simulink model "ASM_Traffic"  (R2026a)
settings: Solver=ode1  StartTime=SIM.tstart.v  StopTime=SIM.tend.v  FixedStep=SIM.StepSize.v
PostLoadFcn:
  | if any(exist('dsrtsu_mdlpostloadfcn', 'file') ~= 0), dsrtsu_mdlpostloadfcn('Execute', bdroot); end
  | try, asm_mdl_postloadfcn(bdroot, 'UpdateModel', 3600); catch, disp(lasterr); end,
InitFcn:
  | , if any(exist('rtifpga_mdlclblib', 'file') ~= 0), rtifpga_mdlclblib('Init', bdroot); end,
  | , if any(exist('dsmpb_private', 'file') ~= 0), dsmpb_private('dsmpb_mdlclblib', 'Init', bdroot); end,
model workspace (MAT data in the model file):
  asmReferencePath = [0 0.01 0.02 0.03 0.04 0.05 0.06 0.07 0.08 0.09 0.1 0.11 ... (350007 elements, 50001x7)]
  roadBounds : Simulink.Parameter (value not decoded)
  safetyAxes : Simulink.Parameter (value not decoded)
undefined symbols (not defined in the file): _to_, a0b2, ASM_BrakeHydraulics_DemoSystems, ASM_VehicleDynamics_DemoSystems, b98103fe8ad365046cd0, BrakeCircuit, controllerConfig, CPT, Crankshaft, DiscIntNeverNeededParam, dsmsi, FinalDriveAssembly, MDL, ModeSignals, mu, Pos_BrakePedal_Maneuver, rad, RefSignals, roadFamilyData, roadFamilyId, s_to_rpm, SIM, SoftECU, Suspension, Tire, Transmission
libraries: ASM_Traffic_lib x135, simulink x98, ASM_Utils_lib x77, ASM_VehicleDynamics_lib x70, ASM_Environment_lib x22, dsmpblib x20, dsmsilib x15, MDLD_Utils_lib x10, ASM_BrakeHydraulics_lib x3, sl_discontinuities x2
(part 11 of 65)

== system ASM_Traffic/DomainControl/DriverAssistance/Interface_In ==
  note: Driver Assistance
  In : Inport
  Bus Creator : BusCreator  Inputs=2
  Bus Selector : BusSelector  OutputSignals=Environment.Plant.Sw_ModelPortBlocks[0Disabled|1Enabled],Environment.Plant.Sw_ModelDeskPlottingInterface[0Disabled|1Enabled],VehicleDynamics.Plant.v_x_Vehicle_CoG[km|h],VehicleDynamics.Plant.YawRate_Vehicle_CoG[deg|s],VehicleDynamics.Plant.Pos_FL_Wheel[x;y;z][m],VehicleDynamics.Plant.Pos_FR_Wheel[x;y;z][m],VehicleDynamics.Plant.r_Dyn_Tire[FL;FR;RL;RR][m],VehicleDynamics.Plant.Coef_RollingRes[FL;FR;RL;RR][],VehicleDynamics.Plant.Cw_x[],VehicleDynamics.Plant.m_TotalVehicle[kg],Drivetrain.Plant.i_FrontDrive[],Drivetrain.Plant.i_RearDrive[],Drivetrain.Plant.TrqDistri_Front_Rear[0_1],Drivetrain.Plant.i_unsync_Trm[],Driver.Plant.Pos_AccPedal[%],Driver.Plant.Pos_BrakePedal[%],Environment.Plant.Slope_Veh_Road[%],Environment.Plant.s_Vehicle_Road[m],Environment.Plant.d_Vehicle_Road[m],Environment.Plant.ECU_Commands[],Environment.Plant.Reset_States[0|1],Environment.Plant.Dist_Fellows[m],Environment.Plant.v_Rel_Fellows[m|s],Environment.Plant.Angle_Hor_Rel_Fellows[deg],Environment.Plant.s_Fellows_Ref[m],Environment.Plant.d_Total_Fellows[m],Environment.Plant.PosVec_MainPnt_Fellows[x;y;z][m],Environment.Plant.Length_Fellows[m],Environment.Plant.Width_Fellows[m],Environment.Plant.Height_Fellows[m],Environment.Plant.Object_ID[],VehicleDynamics.Plant.v_Vehicle[km|h],Engine.Plant.Trq_Fric_Engine[Nm]
  Bus Selector1 : BusSelector  OutputSignals=Environment.Plant.Sw_ModelPortBlocks[0Disabled|1Enabled]
  ExternalSignals : Subsystem
  ModelSignals : Subsystem
  Out : Outport  VectorParamsAs1DForOutWhenUnconnected=off
  wires:
  Bus Selector1/1 -> ExternalSignals/Enable  "<Sw_ModelPortBlocks[0Disabled|1Enabled]>"
  ExternalSignals/1(ExternalECU_ACC_Out) -> Bus Creator/2
  Bus Selector/2 -> ModelSignals/2(Sw_ModelDeskPlottingInterface[0Disabled|1Enabled])  "<Sw_ModelDeskPlottingInterface[0Disabled|1Enabled]>"
  Bus Selector/1 -> ModelSignals/1(Sw_ModelPortBlocks[0Disabled|1Enabled])  "<Sw_ModelPortBlocks[0Disabled|1Enabled]>"
  In/1 -> Bus Selector1/1, Bus Selector/1
  Bus Selector/32 -> ModelSignals/32(v_Vehicle[km|h])  "<v_Vehicle[km|h]>"
  ModelSignals/1(Out) -> Bus Creator/1
  Bus Selector/31 -> ModelSignals/31(Object_ID[])  "<Object_ID[]>"
  Bus Selector/30 -> ModelSignals/30(Height_Fellows[m])  "<Height_Fellows[m]>"
  Bus Selector/29 -> ModelSignals/29(Width_Fellows[m])  "<Width_Fellows[m]>"
  Bus Selector/28 -> ModelSignals/28(Length_Fellows[m])  "<Length_Fellows[m]>"
  Bus Selector/27 -> ModelSignals/27(PosVec_MainPnt_Fellows[x;y;z][m])  "<PosVec_MainPnt_Fellows[x;y;z][m]>"
  Bus Selector/26 -> ModelSignals/26(d_Total_Fellows[m])  "<d_Total_Fellows[m]>"
  Bus Selector/25 -> ModelSignals/25(s_Fellows_Ref[m])  "<s_Fellows_Ref[m]>"
  Bus Selector/24 -> ModelSignals/24(Angle_Hor_Rel_Fellows[deg])  "<Angle_Hor_Rel_Fellows[deg]>"
  Bus Selector/23 -> ModelSignals/23(v_Rel_Fellows[m|s])  "<v_Rel_Fellows[m|s]>"
  Bus Selector/22 -> ModelSignals/22(Dist_Fellows[m])  "<Dist_Fellows[m]>"
  Bus Selector/21 -> ModelSignals/21(Reset[0|1])  "<Reset_States[0|1]>"
  Bus Selector/20 -> ModelSignals/20(ECU_Commands[])  "<ECU_Commands[]>"
  Bus Selector/19 -> ModelSignals/19(d_Vehicle_Road[m])  "<d_Vehicle_Road[m]>"
  Bus Selector/18 -> ModelSignals/18(s_Vehicle_Road[m])  "<s_Vehicle_Road[m]>"
  Bus Selector/17 -> ModelSignals/17(Slope_Veh_Road[%])  "<Slope_Veh_Road[%]>"
  Bus Selector/16 -> ModelSignals/16(Pos_BrakePedal[%])  "<Pos_BrakePedal[%]>"
  Bus Selector/15 -> ModelSignals/15(Pos_AccPedal[%])  "<Pos_AccPedal[%]>"
  Bus Selector/11 -> ModelSignals/11(i_FrontDrive[])  "<i_FrontDrive[]>"
  Bus Selector/10 -> ModelSignals/10(m_TotalVehicle[kg])  "<m_TotalVehicle[kg]>"
  Bus Selector/9 -> ModelSignals/9(Cw_x[])  "<Cw_x[]>"
  Bus Selector/8 -> ModelSignals/8(Coef_RollingRes[FL;FR;RL;RR][])  "<Coef_RollingRes[FL;FR;RL;RR][]>"
  Bus Selector/7 -> ModelSignals/7(r_Dyn_Tire[FL;FR;RL;RR][m])  "<r_Dyn_Tire[FL;FR;RL;RR][m]>"
  Bus Selector/6 -> ModelSignals/6(Pos_FR_Wheel[x;y;z][m])  "<Pos_FR_Wheel[x;y;z][m]>"
  Bus Selector/5 -> ModelSignals/5(Pos_FL_Wheel[x;y;z][m])  "<Pos_FL_Wheel[x;y;z][m]>"
  Bus Selector/4 -> ModelSignals/4(YawRate_Vehicle_CoG[deg|s])  "<YawRate_Vehicle_CoG[deg|s]>"
  Bus Selector/3 -> ModelSignals/3(v_x_Vehicle_CoG[km|h])  "<v_x_Vehicle_CoG[km|h]>"
  Bus Creator/1 -> Out/1
  Bus Selector/14 -> ModelSignals/14(i_unsync_Trm[])  "<i_unsync_Trm[]>"
  Bus Selector/33 -> ModelSignals/33(Trq_Fric_Engine[Nm])  "<Trq_Fric_Engine[Nm]>"
  Bus Selector/12 -> ModelSignals/12(i_RearDrive[])  "<i_RearDrive[]>"
  Bus Selector/13 -> ModelSignals/13(TrqDistri_Front_Rear[0_1][])  "<TrqDistri_Front_Rear[0_1]>"

== system ASM_Traffic/DomainControl/DriverAssistance/Interface_Out ==
  note: Driver Assistance
  In : Inport
  Animation : Subsystem
  Bus Creator1 : BusCreator  Inputs=2
  Bus Selector5 : BusSelector  OutputSignals=SoftECU_ACC.Controller_ACC.State_ACC[0Off|1On],SoftECU_ACC.Target_Selection_ACC.Target_Detected[0|1],SoftECU_ACC.Controller_ACC.v_Set[km|h],SoftECU_ACC.Controller_ACC.Distance_Set[m],SoftECU_ACC.Target_Selection_ACC.Dist_Long[m]
  Bus Selector6 : BusSelector  OutputSignals=ECU_ACC.Enable_Trq_Increase_ACC[0|1],ECU_ACC.Trq_IncreaseRequest_ACC[Nm],ECU_ACC.Trq_IncreaseRequest_ACC[Front;Rear][Nm],ECU_ACC.Enable_Trq_Decrease_ACC[0|1],ECU_ACC.Trq_DecreaseRequest_ACC[Nm],ECU_ACC.AEB[0|1],ECU_ACC.FCW[0|1],ECU_ACC.ACC_State[1OFF|2Standby|3ON],ECU_ACC.Driver_Override_ACC_Active[0Off|1On],ECU_ACC.Driver_Override_ACC_Reason[0NoOverride|1BrakePedal|2AccPedal]
  Control_ModelSignals : Subsystem
  Out : Outport  VectorParamsAs1DForOutWhenUnconnected=off
  wires:
  Bus Selector6/6 -> Control_ModelSignals/6(AEB[0|1])  "<AEB[0|1]>"
  Bus Selector6/7 -> Control_ModelSignals/7(FCW[0|1])  "<FCW[0|1]>"
  Bus Selector6/5 -> Control_ModelSignals/5(Trq_DecreaseRequest_ACC[Nm])  "<Trq_DecreaseRequest_ACC[Nm]>"
  Bus Selector6/4 -> Control_ModelSignals/4(Enable_Trq_Decrease_ACC[0|1])  "<Enable_Trq_Decrease_ACC[0|1]>"
  Bus Selector6/2 -> Control_ModelSignals/2(Trq_IncreaseRequest_ACC[Nm])  "<Trq_IncreaseRequest_ACC[Nm]>"
  Bus Selector6/1 -> Control_ModelSignals/1(Enable_Trq_Increase_ACC[0|1])  "<Enable_Trq_Increase_ACC[0|1]>"
  In/1 -> Bus Selector5/1, Bus Selector6/1
  Bus Selector6/3 -> Control_ModelSignals/3(Trq_IncreaseRequest_ACC[Front;Rear][Nm])  "<Trq_IncreaseRequest_ACC[Front;Rear][Nm]>"
  Bus Creator1/1 -> Out/1  "DriverAssistance"
  Control_ModelSignals/1(Out) -> Bus Creator1/1
  Animation/1(Out) -> Bus Creator1/2
  Bus Selector5/1 -> Animation/1(State_ACC[0Off|1On])  "<State_ACC[0Off|1On]>"
  Bus Selector5/2 -> Animation/2(Target_Detected[0|1])  "<Target_Detected[0|1]>"
  Bus Selector5/3 -> Animation/3(v_Set[km|h])  "<v_Set[km|h]>"
  Bus Selector5/4 -> Animation/4(Distance_Set[m])  "<Distance_Set[m]>"
  Bus Selector5/5 -> Animation/5(Dist_Long[m])  "<Dist_Long[m]>"
  Bus Selector6/8 -> Control_ModelSignals/8(ACC_State[1OFF|2Standby|3ON])  "<ACC_State[1OFF|2Standby|3ON]>"
  Bus Selector6/9 -> Control_ModelSignals/9(Driver_Override_ACC_Active[0Off|1On])  "<Driver_Override_ACC_Active[0Off|1On]>"
  Bus Selector6/10 -> Control_ModelSignals/10(Driver_Override_ACC_Reason[0NoOverride|1BrakePedal|2AccPedal])  "<Driver_Override_ACC_Reason[0NoOverride|1BrakePedal|2AccPedal]>"

== system ASM_Traffic/DomainControl/DriverAssistance/SignalInterface ==
  In : Inport
  ASMSignalInterface : Subsystem  mask(ASM_SIGNAL_INTERFACE){LabelTextfield=DriverAssistance}
      mask prompts: LabelTextfield "Label"
      mask help:
      | The ASMSignalInterface block processes the ASMSignalBus and provides a vector-based interface for each signal (e.g. ModelDesk Plotting).
      |
      | Always push the update button after you have changed the signal bus structure in order to synchronize the signal interface. The update may take a few seconds.
      | A modified model must be reloaded in ModelDesk to keep consistency of ModelDesk and simulation model plot signals. Therefore select ''Update Model'' from the ''Simulation Model'' context menu of the ModelDesk Project Navigator.
      settings: AttributesFormatString=Label: %<LabelTextfield>
      settings: CopyFcn=|
      | try
      |  set_param(gcb,'LinkStatus', 'none')
      | catch
      | end
      mask Help: eval(['asm_modelhelp(gcbh,''tool'',''ASM_Utils_lib'', ''ASMSIGNALINTERFACE'')'])
      mask DialogControl Hint Prompt: For changes of Label first apply change and then push "Update".
      mask DialogControl UpdateButton Prompt: Update
      mask DialogControl UpdateButton Callback: asm_mdld_plot_block_update(bdroot(gcb), 'update', 'current');
      mask DialogControl UpdateAllButton Prompt: Update All
      mask DialogControl UpdateAllButton Callback: asm_mdld_plot_block_update(bdroot(gcb), 'update', 'all');
  Bus Selector Disable Signals : BusSelector  OutputSignals=ExternalModel.Sw_ModelPortBlocks[0Disabled|1Enabled],ExternalModel.Sw_ModelDeskPlottingInterface[0Disabled|1Enabled]
  ExternalOutports : Subsystem  TreatAsAtomicUnit=on
  wires:
  Bus Selector Disable Signals/2 -> ASMSignalInterface/Enable  "<Sw_ModelDeskPlottingInterface[0Disabled|1Enabled]>"
  Bus Selector Disable Signals/1 -> ExternalOutports/Enable  "<Sw_ModelPortBlocks[0Disabled|1Enabled]>"
  In/1 -> Bus Selector Disable Signals/1
  [ASMBUS_DriverAssistance_Control] -> ASMSignalInterface/1(ASMSignalBus), ExternalOutports/1(In1)

== system ASM_Traffic/DomainControl/StartSystem/Control ==
  note: Start System
  Interface_In : Inport
  SoftECU_StartSystem : Subsystem
  Sw_ECU_Signals : Subsystem
  UserInterface : Subsystem
  Control : Outport  VectorParamsAs1DForOutWhenUnconnected=off
  wires:
  SoftECU_StartSystem/1(ASMSignalBus) -> UserInterface/2(In)
  UserInterface/1(Out) -> SoftECU_StartSystem/1(UserInterface)
  Interface_In/1 -> Sw_ECU_Signals/2(ExternalECU), SoftECU_StartSystem/2(Interface_In), UserInterface/1(Interface_In)
  Sw_ECU_Signals/1(ECU_Signals) -> Control/1
  SoftECU_StartSystem/2(Out) -> Sw_ECU_Signals/1(SoftECU)

== system ASM_Traffic/DomainControl/StartSystem/Interface_In ==
  note: Start System
  In : Inport
  Bus Creator : BusCreator  Inputs=2
  Bus Selector2 : BusSelector  OutputSignals=Environment.Plant.Sw_ModelPortBlocks[0Disabled|1Enabled],Environment.Plant.Sw_ModelDeskPlottingInterface[0Disabled|1Enabled],Driver.Plant.Pos_BrakePedal[%],Driver.Plant.Pos_ClutchPedal[%],Driver.Plant.SelectorLever[-3T|-2P|-1R|0N|1D],Environment.Plant.Reset_States[0|1],Environment.Plant.Sw_StartButton[0Off|1On],DomainControl.TorqueManager.Control.State_Engine[0|1|2|3|4],Environment.Plant.State_StartButton[-1PowerOff|0Acc|1PowerOn|2StarterOn],Drivetrain.Plant.Mode_Transmission[1Manual|2Automatic],Drivetrain.Plant.Sw_CrankShaft_Reset[0Disabled|1Enabled],Environment.Plant.Mode_StartButtonState[1Stim|2SoftECU]
  Bus Selector21 : BusSelector  OutputSignals=Environment.Plant.Sw_ModelPortBlocks[0Disabled|1Enabled]
  ExternalSignals : Subsystem
  ModelSignals : Subsystem
  Out : Outport  VectorParamsAs1DForOutWhenUnconnected=off
  wires:
  Bus Selector21/1 -> ExternalSignals/Enable  "<Sw_ModelPortBlocks[0Disabled|1Enabled]>"
  ExternalSignals/1(ExternalECU_StartSystem_Out) -> Bus Creator/2
  Bus Selector2/2 -> ModelSignals/2(Sw_ModelDeskPlottingInterface[0Disabled|1Enabled])  "<Sw_ModelDeskPlottingInterface[0Disabled|1Enabled]>"
  Bus Selector2/1 -> ModelSignals/1(Sw_ModelPortBlocks[0Disabled|1Enabled])  "<Sw_ModelPortBlocks[0Disabled|1Enabled]>"
  In/1 -> Bus Selector21/1, Bus Selector2/1
  Bus Selector2/7 -> ModelSignals/7(Sw_StartButton[0Off|1On])  "<Sw_StartButton[0Off|1On]>"
  Bus Creator/1 -> Out/1
  Bus Selector2/6 -> ModelSignals/6(Reset_States[0|1])  "<Reset_States[0|1]>"
  Bus Selector2/5 -> ModelSignals/5(SelectorLever[-3T|-2P|-1R|0N|1D])  "<SelectorLever[-3T|-2P|-1R|0N|1D]>"
  Bus Selector2/3 -> ModelSignals/3(Pos_BrakePedal[%])  "<Pos_BrakePedal[%]>"
  Bus Selector2/4 -> ModelSignals/4(Pos_ClutchPedal[%])  "<Pos_ClutchPedal[%]>"
  Bus Selector2/8 -> ModelSignals/8(State_Engine[0|1|2|3|4])  "<State_Engine[0|1|2|3|4]>"
  Bus Selector2/9 -> ModelSignals/9(State_StartButton[-1PowerOff|0Acc|1PowerOn|2StarterOn])  "<State_StartButton[-1PowerOff|0Acc|1PowerOn|2StarterOn]>"
  Bus Selector2/10 -> ModelSignals/10(Mode_Transmission[1Manual|2Automatic])  "<Mode_Transmission[1Manual|2Automatic]>"
  Bus Selector2/11 -> ModelSignals/11(Sw_CrankShaft_Reset[0Disabled|1Enabled])  "<Sw_CrankShaft_Reset[0Disabled|1Enabled]>"
  Bus Selector2/12 -> ModelSignals/12(Mode_StartButtonState[1Stim|2SoftECU])  "<Mode_StartButtonState[1Stim|2SoftECU]>"
  ModelSignals/1(Out) -> Bus Creator/1

== system ASM_Traffic/DomainControl/StartSystem/Interface_Out ==
  note: Start System
  In : Inport
  Bus Creator1 : BusCreator  Inputs=1
  Bus Selector1 : BusSelector  OutputSignals=State_StartButton[-2|-1|0|1|2|3],Sw_Ignition[0|1],Sw_StarterReq[0|1]
  Control_ModelSignals : Subsystem
  Out : Outport  VectorParamsAs1DForOutWhenUnconnected=off
  wires:
  In/1 -> Bus Selector1/1
  Bus Selector1/2 -> Control_ModelSignals/2(Sw_Ignition[0|1])  "<Sw_Ignition[0|1]>"
  Bus Selector1/3 -> Control_ModelSignals/3(Sw_StarterReq[0|1])  "<Sw_StarterReq[0|1]>"
  Bus Creator1/1 -> Out/1  "StartSystem"
  Control_ModelSignals/1(Out) -> Bus Creator1/1
  Bus Selector1/1 -> Control_ModelSignals/1(State_StartButton[-2|-1|0|1|2|3])  "<State_StartButton[-2|-1|0|1|2|3]>"

== system ASM_Traffic/DomainControl/StartSystem/SignalInterface ==
  In : Inport
  ASMSignalInterface : Subsystem  mask(ASM_SIGNAL_INTERFACE){LabelTextfield=StartSystem}
      mask prompts: LabelTextfield "Label"
      mask help:
      | The ASMSignalInterface block processes the ASMSignalBus and provides a vector-based interface for each signal (e.g. ModelDesk Plotting).
      |
      | Always push the update button after you have changed the signal bus structure in order to synchronize the signal interface. The update may take a few seconds.
      | A modified model must be reloaded in ModelDesk to keep consistency of ModelDesk and simulation model plot signals. Therefore select ''Update Model'' from the ''Simulation Model'' context menu of the ModelDesk Project Navigator.
      settings: AttributesFormatString=Label: %<LabelTextfield>
      settings: CopyFcn=|
      | try
      |  set_param(gcb,'LinkStatus', 'none')
      | catch
      | end
      mask Help: eval(['asm_modelhelp(gcbh,''tool'',''ASM_Utils_lib'', ''ASMSIGNALINTERFACE'')'])
      mask DialogControl Hint Prompt: For changes of Label first apply change and then push "Update".
      mask DialogControl UpdateButton Prompt: Update
      mask DialogControl UpdateButton Callback: asm_mdld_plot_block_update(bdroot(gcb), 'update', 'current');
      mask DialogControl UpdateAllButton Prompt: Update All
      mask DialogControl UpdateAllButton Callback: asm_mdld_plot_block_update(bdroot(gcb), 'update', 'all');
  Bus Selector Disable Signals : BusSelector  OutputSignals=ExternalModel.Sw_ModelPortBlocks[0Disabled|1Enabled],ExternalModel.Sw_ModelDeskPlottingInterface[0Disabled|1Enabled]
  ExternalOutports : Subsystem  TreatAsAtomicUnit=on
  wires:
  Bus Selector Disable Signals/2 -> ASMSignalInterface/Enable  "<Sw_ModelDeskPlottingInterface[0Disabled|1Enabled]>"
  Bus Selector Disable Signals/1 -> ExternalOutports/Enable  "<Sw_ModelPortBlocks[0Disabled|1Enabled]>"
  In/1 -> Bus Selector Disable Signals/1
  [ASMBUS_StartSystem_Control] -> ASMSignalInterface/1(ASMSignalBus), ExternalOutports/1(In1)

== system ASM_Traffic/DomainControl/TorqueManager/Control ==
  note: Torque Manager Basic
  Interface_In : Inport
  SoftECU_TorqueManager : Subsystem
  UserInterface : Subsystem
  Control : Outport  VectorParamsAs1DForOutWhenUnconnected=off
  wires:
  SoftECU_TorqueManager/1(ASMSignalBus) -> UserInterface/1(In)
  UserInterface/1(Out) -> SoftECU_TorqueManager/1(UserInterface)
  Interface_In/1 -> SoftECU_TorqueManager/2(Interface_In)
  SoftECU_TorqueManager/2(Out) -> Control/1

== system ASM_Traffic/DomainControl/TorqueManager/Interface_In ==
  note: Torque Manager Basic
  In : Inport
  Bus Creator : BusCreator  Inputs=1
  Bus Selector2 : BusSelector  OutputSignals=Environment.Plant.Sw_ModelPortBlocks[0Disabled|1Enabled],Environment.Plant.Sw_ModelDeskPlottingInterface[0Disabled|1Enabled],Driver.Plant.Pos_BrakePedal[%],Engine.Control.State_ICEngine[0|1|2|3|4],DomainControl.StartSystem.Control.Sw_Ignition[0|1],DomainControl.StartSystem.Control.Sw_StarterReq[0|1],Engine.Control.Sw_Starter[0Off|1On]
  ModelSignals : Subsystem
  Out : Outport  VectorParamsAs1DForOutWhenUnconnected=off
  wires:
  Bus Selector2/2 -> ModelSignals/2(Sw_ModelDeskPlottingInterface[0Disabled|1Enabled])  "<Sw_ModelDeskPlottingInterface[0Disabled|1Enabled]>"
  Bus Selector2/1 -> ModelSignals/1(Sw_ModelPortBlocks[0Disabled|1Enabled])  "<Sw_ModelPortBlocks[0Disabled|1Enabled]>"
  In/1 -> Bus Selector2/1
  Bus Selector2/4 -> ModelSignals/4(State_Engine[0|1|2|3|4])  "<State_ICEngine[0|1|2|3|4]>"
  Bus Selector2/3 -> ModelSignals/3(Pos_BrakePedal[%])  "<Pos_BrakePedal[%]>"
  ModelSignals/1(Out) -> Bus Creator/1
  Bus Creator/1 -> Out/1
  Bus Selector2/5 -> ModelSignals/5(Sw_Ignition[0|1])  "<Sw_Ignition[0|1]>"
  Bus Selector2/6 -> ModelSignals/6(Sw_StarterReq[0|1])  "<Sw_StarterReq[0|1]>"
  Bus Selector2/7 -> ModelSignals/7(Sw_Starter[0Off|1On])  "<Sw_Starter[0Off|1On]>"

== system ASM_Traffic/DomainControl/TorqueManager/Interface_Out ==
  note: Torque Manager Basic
  In : Inport
  " Mode_BSG[-1|0|1|2|3|4|5]" : Constant  Value=-1
  Bus Creator1 : BusCreator  Inputs=1
  Bus Selector : BusSelector  OutputSignals=ExternalModel.Sw_Ignition[0|1],ExternalModel.Sw_StarterReq[0|1],ExternalModel.Pos_BrakePedal[%],ExternalModel.Sw_Starter[0Off|1On],ExternalModel.State_Engine[0|1|2|3|4]
  Control_ModelSignals : Subsystem
  HybridMode_ICE[0Off|1OnIdle|2OnPower|3err] : Constant  Value=0
  Sw_DriveMode[0Hybrid|1ICE|2EM] : Constant
  Trq_Request_Brake[Nm] : Constant  Value=0
  Trq_Request_EM[Nm] : Constant  Value=0
  Trq_Request_ICE[Nm] : Constant  Value=-9000
  Vehicle_Topology[-2|-1|0|2] : Constant  Value=-1
  Out : Outport  VectorParamsAs1DForOutWhenUnconnected=off
  wires:
  HybridMode_ICE[0Off|1OnIdle|2OnPower|3err]/1 -> Control_ModelSignals/9(HybridMode_ICE[0Off|1OnIdle|2OnPower|3err])
  Trq_Request_ICE[Nm]/1 -> Control_ModelSignals/8(Trq_Request_ICE[Nm])
  Sw_DriveMode[0Hybrid|1ICE|2EM]/1 -> Control_ModelSignals/11(Sw_DriveMode[0Hybrid|1ICE|2EM])
  In/1 -> Bus Selector/1
  Control_ModelSignals/1(Out) -> Bus Creator1/1
  Bus Selector/1 -> Control_ModelSignals/1(Ignition_ICE[0Off|1On])  "<Sw_Ignition[0|1]>"
  Bus Selector/2 -> Control_ModelSignals/2(StarterReq_ICE[0Off|1On])  "<Sw_StarterReq[0|1]>"
  Bus Selector/3 -> Control_ModelSignals/3(Pos_BrakePedal_Desired[%])  "<Pos_BrakePedal[%]>"
  Trq_Request_EM[Nm]/1 -> Control_ModelSignals/7(Trq_Request_EM[Nm])
  " Mode_BSG[-1|0|1|2|3|4|5]"/1 -> Control_ModelSignals/6(" Mode_BSG[-1|0|1|2|3|4|5]")
  Bus Selector/4 -> Control_ModelSignals/4(Starter_Drivetrain[0Off|1On])  "<Sw_Starter[0Off|1On]>"
  Trq_Request_Brake[Nm]/1 -> Control_ModelSignals/10(Trq_Request_Brake[Nm])
  Vehicle_Topology[-2|-1|0|2]/1 -> Control_ModelSignals/12(Vehicle_Topology[-2|-1|0|2])
  Bus Creator1/1 -> Out/1  "TorqueManager"
  Bus Selector/5 -> Control_ModelSignals/5(State_Engine[0|1|2|3|4])  "<State_Engine[0|1|2|3|4]>"

== system ASM_Traffic/DomainControl/TorqueManager/SignalInterface ==
  In : Inport
  ASMSignalInterface : Subsystem  mask(ASM_SIGNAL_INTERFACE){LabelTextfield=TorqueManager}
      mask prompts: LabelTextfield "Label"
      mask help:
      | The ASMSignalInterface block processes the ASMSignalBus and provides a vector-based interface for each signal (e.g. ModelDesk Plotting).
      |
      | Always push the update button after you have changed the signal bus structure in order to synchronize the signal interface. The update may take a few seconds.
      | A modified model must be reloaded in ModelDesk to keep consistency of ModelDesk and simulation model plot signals. Therefore select ''Update Model'' from the ''Simulation Model'' context menu of the ModelDesk Project Navigator.
      settings: AttributesFormatString=Label: %<LabelTextfield>
      settings: CopyFcn=|
      | try
      |  set_param(gcb,'LinkStatus', 'none')
      | catch
      | end
      mask Help: eval(['asm_modelhelp(gcbh,''tool'',''ASM_Utils_lib'', ''ASMSIGNALINTERFACE'')'])
      mask DialogControl Hint Prompt: For changes of Label first apply change and then push "Update".
      mask DialogControl UpdateButton Prompt: Update
      mask DialogControl UpdateButton Callback: asm_mdld_plot_block_update(bdroot(gcb), 'update', 'current');
      mask DialogControl UpdateAllButton Prompt: Update All
      mask DialogControl UpdateAllButton Callback: asm_mdld_plot_block_update(bdroot(gcb), 'update', 'all');
  Bus Selector Disable Signals : BusSelector  OutputSignals=ExternalModel.Sw_ModelPortBlocks[0Disabled|1Enabled],ExternalModel.Sw_ModelDeskPlottingInterface[0Disabled|1Enabled]
  ExternalOutports : Subsystem  TreatAsAtomicUnit=on
  wires:
  Bus Selector Disable Signals/2 -> ASMSignalInterface/Enable  "<Sw_ModelDeskPlottingInterface[0Disabled|1Enabled]>"
  Bus Selector Disable Signals/1 -> ExternalOutports/Enable  "<Sw_ModelPortBlocks[0Disabled|1Enabled]>"
  In/1 -> Bus Selector Disable Signals/1
  [ASMBUS_TorqueManager_Control] -> ExternalOutports/1(In1), ASMSignalInterface/1(ASMSignalBus)

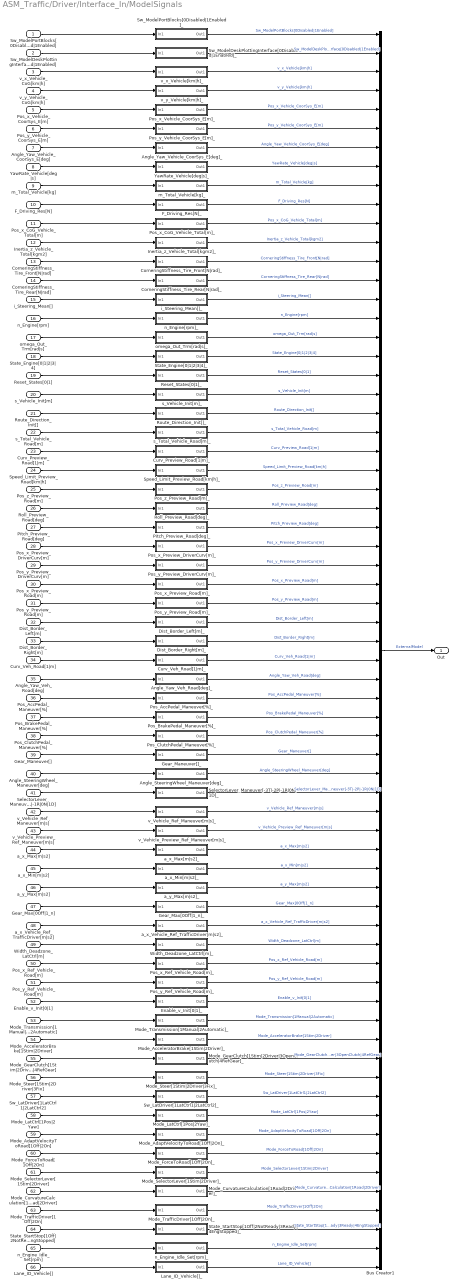
== system ASM_Traffic/Driver/Interface_In/ModelSignals ==
  Sw_ModelPortBlocks[0Disabled|1Enabled] : Inport
  Sw_ModelDeskPlottingInterface[0Disabled|1Enabled] : Inport  Port=2
  v_x_Vehicle_CoG[km|h] : Inport  Port=3
  v_y_Vehicle_CoG[km|h] : Inport  Port=4
  Pos_x_Vehicle_CoorSys_E[m] : Inport  Port=5
  Pos_y_Vehicle_CoorSys_E[m] : Inport  Port=6
  Angle_Yaw_Vehicle_CoorSys_E[deg] : Inport  Port=7
  YawRate_Vehicle[deg|s] : Inport  Port=8
  m_Total_Vehicle[kg] : Inport  Port=9
  F_Driving_Res[N] : Inport  Port=10
  Pos_x_CoG_Vehicle_Total[m] : Inport  Port=11
  Inertia_z_Vehicle_Total[kgm2] : Inport  Port=12
  CorneringStiffness_Tire_Front[N|rad] : Inport  Port=13
  CorneringStiffness_Tire_Rear[N|rad] : Inport  Port=14
  i_Steering_Mean[] : Inport  Port=15
  n_Engine[rpm] : Inport  Port=16
  omega_Out_Trm[rad|s] : Inport  Port=17
  State_Engine[0|1|2|3|4] : Inport  Port=18
  Reset_States[0|1] : Inport  Port=19
  s_Vehicle_Init[m] : Inport  Port=20
  Route_Direction_Init[] : Inport  Port=21
  s_Total_Vehicle_Road[m] : Inport  Port=22
  Curv_Preview_Road[1|m] : Inport  Port=23
  Speed_Limit_Preview_Road[km|h] : Inport  Port=24
  Pos_z_Preview_Road[m] : Inport  Port=25
  Roll_Preview_Road[deg] : Inport  Port=26
  Pitch_Preview_Road[deg] : Inport  Port=27
  Pos_x_Preview_DriverCurv[m] : Inport  Port=28
  Pos_y_Preview_DriverCurv[m] : Inport  Port=29
  Pos_x_Preview_Road[m] : Inport  Port=30
  Pos_y_Preview_Road[m] : Inport  Port=31
  Dist_Border_Left[m] : Inport  Port=32
  Dist_Border_Right[m] : Inport  Port=33
  Curv_Veh_Road[1|m] : Inport  Port=34
  Angle_Yaw_Veh_Road[deg] : Inport  Port=35
  Pos_AccPedal_Maneuver[%] : Inport  Port=36
  Pos_BrakePedal_Maneuver[%] : Inport  Port=37
  Pos_ClutchPedal_Maneuver[%] : Inport  Port=38
  Gear_Maneuver[] : Inport  Port=39
  Angle_SteeringWheel_Maneuver[deg] : Inport  Port=40
  SelectorLever_Maneuver[-3T|-2P|-1R|0N|1D] : Inport  Port=41
  v_Vehicle_Ref_Maneuver[m|s] : Inport  Port=42
  v_Vehicle_Preview_Ref_Maneuver[m|s] : Inport  Port=43
  a_x_Max[m|s2] : Inport  Port=44
  a_x_Min[m|s2] : Inport  Port=45
  a_y_Max[m|s2] : Inport  Port=46
  Gear_Max[0Off|1_n] : Inport  Port=47
  a_x_Vehicle_Ref_TrafficDriver[m|s2] : Inport  Port=48
  Width_Deadzone_LatCtrl[m] : Inport  Port=49
  Pos_x_Ref_Vehicle_Road[m] : Inport  Port=50
  Pos_y_Ref_Vehicle_Road[m] : Inport  Port=51
  Enable_v_Init[0|1] : Inport  Port=52
  Mode_Transmission[1Manual|2Automatic] : Inport  Port=53
  Mode_AcceleratorBrake[1Stim|2Driver] : Inport  Port=54
  Mode_GearClutch[1Stim|2Driver|3OpenClutch|4RefGear] : Inport  Port=55
  Mode_Steer[1Stim|2Driver|3Fix] : Inport  Port=56
  Sw_LatDriver[1LatCtrl1|2LatCtrl2] : Inport  Port=57
  Mode_LatCtrl[1Pos|2Yaw] : Inport  Port=58
  Mode_AdaptVelocityToRoad[1Off|2On] : Inport  Port=59
  Mode_ForceToRoad[1Off|2On] : Inport  Port=60
  Mode_SelectorLever[1Stim|2Driver] : Inport  Port=61
  Mode_CurvatureCalculation[1Road|2Driver] : Inport  Port=62
  Mode_TrafficDriver[1Off|2On] : Inport  Port=63
  State_StartStop[1Off|2NotReady|3Ready|4EngStopped] : Inport  Port=64
  n_Engine_Idle_Set[rpm] : Inport  Port=65
  Lane_ID_Vehicle[] : Inport  Port=66
  Angle_SteeringWheel_Maneuver[deg]_ : Subsystem
      mask Display: disp('')
  Angle_Yaw_Veh_Road[deg]_ : Subsystem
      mask Display: disp('')
  Angle_Yaw_Vehicle_CoorSys_E[deg]_ : Subsystem
      mask Display: disp('')
  Bus Creator1 : BusCreator  Inputs=66
  CorneringStiffness_Tire_Front[N|rad]_ : Subsystem
      mask Display: disp('')
  CorneringStiffness_Tire_Rear[N|rad]_ : Subsystem
      mask Display: disp('')
  Curv_Preview_Road[1|m]_ : Subsystem
      mask Display: disp('')
  Curv_Veh_Road[1|m]_ : Subsystem
      mask Display: disp('')
  Dist_Border_Left[m]_ : Subsystem
      mask Display: disp('')
  Dist_Border_Right[m]_ : Subsystem
      mask Display: disp('')
  Enable_v_Init[0|1]_ : Subsystem
      mask Display: disp('')
  F_Driving_Res[N]_ : Subsystem
      mask Display: disp('')
  Gear_Maneuver[]_ : Subsystem
      mask Display: disp('')
  Gear_Max[0Off|1_n]_ : Subsystem
      mask Display: disp('')
  Inertia_z_Vehicle_Total[kgm2]_ : Subsystem
      mask Display: disp('')
  Lane_ID_Vehicle[]_ : Subsystem
      mask Display: disp('')
  Mode_AcceleratorBrake[1Stim|2Driver]_ : Subsystem
      mask Display: disp('')
  Mode_AdaptVelocityToRoad[1Off|2On]_ : Subsystem
      mask Display: disp('')
  Mode_CurvatureCalculation[1Road|2Driver]_ : Subsystem
      mask Display: disp('')
  Mode_ForceToRoad[1Off|2On]_ : Subsystem
      mask Display: disp('')
  Mode_GearClutch[1Stim|2Driver|3OpenClutch|4RefGear]_ : Subsystem
      mask Display: disp('')
  Mode_LatCtrl[1Pos|2Yaw]_ : Subsystem
      mask Display: disp('')
  Mode_SelectorLever[1Stim|2Driver]_ : Subsystem
      mask Display: disp('')
  Mode_Steer[1Stim|2Driver|3Fix]_ : Subsystem
      mask Display: disp('')
  Mode_TrafficDriver[1Off|2On]_ : Subsystem
      mask Display: disp('')
  Mode_Transmission[1Manual|2Automatic]_ : Subsystem
      mask Display: disp('')
  Pitch_Preview_Road[deg]_ : Subsystem
      mask Display: disp('')
  Pos_AccPedal_Maneuver[%]_ : Subsystem
      mask Display: disp('')
  Pos_BrakePedal_Maneuver[%]_ : Subsystem
      mask Display: disp('')
  Pos_ClutchPedal_Maneuver[%]_ : Subsystem
      mask Display: disp('')
  Pos_x_CoG_Vehicle_Total[m]_ : Subsystem
      mask Display: disp('')
  Pos_x_Preview_DriverCurv[m]_ : Subsystem
      mask Display: disp('')
  Pos_x_Preview_Road[m]_ : Subsystem
      mask Display: disp('')
  Pos_x_Ref_Vehicle_Road[m]_ : Subsystem
      mask Display: disp('')
  Pos_x_Vehicle_CoorSys_E[m]_ : Subsystem
      mask Display: disp('')
  Pos_y_Preview_DriverCurv[m]_ : Subsystem
      mask Display: disp('')
  Pos_y_Preview_Road[m]_ : Subsystem
      mask Display: disp('')
  Pos_y_Ref_Vehicle_Road[m]_ : Subsystem
      mask Display: disp('')
  Pos_y_Vehicle_CoorSys_E[m]_ : Subsystem
      mask Display: disp('')
  Pos_z_Preview_Road[m]_ : Subsystem
      mask Display: disp('')
  Reset_States[0|1]_ : Subsystem
      mask Display: disp('')
  Roll_Preview_Road[deg]_ : Subsystem
      mask Display: disp('')
  Route_Direction_Init[]_ : Subsystem
      mask Display: disp('')
  SelectorLever_Maneuver[-3T|-2P|-1R|0N|1D]_ : Subsystem
      mask Display: disp('')
  Speed_Limit_Preview_Road[km|h]_ : Subsystem
      mask Display: disp('')
  State_Engine[0|1|2|3|4]_ : Subsystem
      mask Display: disp('')
  State_StartStop[1Off|2NotReady|3Ready|4EngStopped]_ : Subsystem
      mask Display: disp('')
  Sw_LatDriver[1LatCtrl1|2LatCtrl2]_ : Subsystem
      mask Display: disp('')
  Sw_ModelDeskPlottingInterface[0Disabled|1Enabled]_ : Subsystem
  Sw_ModelPortBlocks[0Disabled|1Enabled]_ : Subsystem
  Width_Deadzone_LatCtrl[m]_ : Subsystem
      mask Display: disp('')
  YawRate_Vehicle[deg|s]_ : Subsystem
      mask Display: disp('')
  a_x_Max[m|s2]_ : Subsystem
      mask Display: disp('')
  a_x_Min[m|s2]_ : Subsystem
      mask Display: disp('')
  a_x_Vehicle_Ref_TrafficDriver[m|s2]_ : Subsystem
      mask Display: disp('')
  a_y_Max[m|s2]_ : Subsystem
      mask Display: disp('')
  i_Steering_Mean[]_ : Subsystem
      mask Display: disp('')
  m_Total_Vehicle[kg]_ : Subsystem
      mask Display: disp('')
  n_Engine[rpm]_ : Subsystem
      mask Display: disp('')
  n_Engine_Idle_Set[rpm]_ : Subsystem
      mask Display: disp('')
  omega_Out_Trm[rad|s]_ : Subsystem
      mask Display: disp('')
  s_Total_Vehicle_Road[m]_ : Subsystem
      mask Display: disp('')
  s_Vehicle_Init[m]_ : Subsystem
      mask Display: disp('')
  v_Vehicle_Preview_Ref_Maneuver[m|s]_ : Subsystem
      mask Display: disp('')
  v_Vehicle_Ref_Maneuver[m|s]_ : Subsystem
      mask Display: disp('')
  v_x_Vehicle[km|h]_ : Subsystem
      mask Display: disp('')
  v_y_Vehicle[km|h]_ : Subsystem
      mask Display: disp('')
  Out : Outport  VectorParamsAs1DForOutWhenUnconnected=off
  wires:
  Sw_ModelDeskPlottingInterface[0Disabled|1Enabled]_/1(Out1) -> Bus Creator1/2  "Sw_ModelDeskPlottingInterface[0Disabled|1Enabled]"
  Sw_ModelPortBlocks[0Disabled|1Enabled]_/1(Out1) -> Bus Creator1/1  "Sw_ModelPortBlocks[0Disabled|1Enabled]"
  Sw_ModelDeskPlottingInterface[0Disabled|1Enabled]/1 -> Sw_ModelDeskPlottingInterface[0Disabled|1Enabled]_/1(In1)
  Sw_ModelPortBlocks[0Disabled|1Enabled]/1 -> Sw_ModelPortBlocks[0Disabled|1Enabled]_/1(In1)
  Bus Creator1/1 -> Out/1  "ExternalModel"
  Pos_AccPedal_Maneuver[%]_/1(Out1) -> Bus Creator1/36  "Pos_AccPedal_Maneuver[%]"
  Pos_BrakePedal_Maneuver[%]/1 -> Pos_BrakePedal_Maneuver[%]_/1(In1)
  v_Vehicle_Preview_Ref_Maneuver[m|s]/1 -> v_Vehicle_Preview_Ref_Maneuver[m|s]_/1(In1)
  Pos_ClutchPedal_Maneuver[%]/1 -> Pos_ClutchPedal_Maneuver[%]_/1(In1)
  SelectorLever_Maneuver[-3T|-2P|-1R|0N|1D]/1 -> SelectorLever_Maneuver[-3T|-2P|-1R|0N|1D]_/1(In1)
  Angle_SteeringWheel_Maneuver[deg]/1 -> Angle_SteeringWheel_Maneuver[deg]_/1(In1)
  Gear_Max[0Off|1_n]/1 -> Gear_Max[0Off|1_n]_/1(In1)
  Pos_ClutchPedal_Maneuver[%]_/1(Out1) -> Bus Creator1/38  "Pos_ClutchPedal_Maneuver[%]"
  SelectorLever_Maneuver[-3T|-2P|-1R|0N|1D]_/1(Out1) -> Bus Creator1/41  "SelectorLever_Maneuver[-3T|-2P|-1R|0N|1D]"
  Angle_SteeringWheel_Maneuver[deg]_/1(Out1) -> Bus Creator1/40  "Angle_SteeringWheel_Maneuver[deg]"
  v_Vehicle_Preview_Ref_Maneuver[m|s]_/1(Out1) -> Bus Creator1/43  "v_Vehicle_Preview_Ref_Maneuver[m|s]"
  Gear_Max[0Off|1_n]_/1(Out1) -> Bus Creator1/47  "Gear_Max[0Off|1_n]"
  Pos_BrakePedal_Maneuver[%]_/1(Out1) -> Bus Creator1/37  "Pos_BrakePedal_Maneuver[%]"
  a_x_Max[m|s2]_/1(Out1) -> Bus Creator1/44  "a_x_Max[m|s2]"
  a_x_Min[m|s2]/1 -> a_x_Min[m|s2]_/1(In1)
  a_y_Max[m|s2]_/1(Out1) -> Bus Creator1/46  "a_y_Max[m|s2]"
  a_x_Min[m|s2]_/1(Out1) -> Bus Creator1/45  "a_x_Min[m|s2]"
  Width_Deadzone_LatCtrl[m]/1 -> Width_Deadzone_LatCtrl[m]_/1(In1)
  Gear_Maneuver[]_/1(Out1) -> Bus Creator1/39  "Gear_Maneuver[]"
  a_y_Max[m|s2]/1 -> a_y_Max[m|s2]_/1(In1)
  Gear_Maneuver[]/1 -> Gear_Maneuver[]_/1(In1)
  v_Vehicle_Ref_Maneuver[m|s]/1 -> v_Vehicle_Ref_Maneuver[m|s]_/1(In1)
  a_x_Vehicle_Ref_TrafficDriver[m|s2]/1 -> a_x_Vehicle_Ref_TrafficDriver[m|s2]_/1(In1)
  Pos_AccPedal_Maneuver[%]/1 -> Pos_AccPedal_Maneuver[%]_/1(In1)
  a_x_Vehicle_Ref_TrafficDriver[m|s2]_/1(Out1) -> Bus Creator1/48  "a_x_Vehicle_Ref_TrafficDriver[m|s2]"
  Width_Deadzone_LatCtrl[m]_/1(Out1) -> Bus Creator1/49  "Width_Deadzone_LatCtrl[m]"
  a_x_Max[m|s2]/1 -> a_x_Max[m|s2]_/1(In1)
  Pos_y_Ref_Vehicle_Road[m]_/1(Out1) -> Bus Creator1/51  "Pos_y_Ref_Vehicle_Road[m]"
  v_Vehicle_Ref_Maneuver[m|s]_/1(Out1) -> Bus Creator1/42  "v_Vehicle_Ref_Maneuver[m|s]"
  Pos_x_Ref_Vehicle_Road[m]/1 -> Pos_x_Ref_Vehicle_Road[m]_/1(In1)
  Pos_x_Ref_Vehicle_Road[m]_/1(Out1) -> Bus Creator1/50  "Pos_x_Ref_Vehicle_Road[m]"
  Pos_y_Ref_Vehicle_Road[m]/1 -> Pos_y_Ref_Vehicle_Road[m]_/1(In1)
  Pos_y_Vehicle_CoorSys_E[m]/1 -> Pos_y_Vehicle_CoorSys_E[m]_/1(In1)
  F_Driving_Res[N]_/1(Out1) -> Bus Creator1/10  "F_Driving_Res[N]"
  m_Total_Vehicle[kg]_/1(Out1) -> Bus Creator1/9  "m_Total_Vehicle[kg]"
  Angle_Yaw_Vehicle_CoorSys_E[deg]/1 -> Angle_Yaw_Vehicle_CoorSys_E[deg]_/1(In1)
  Pos_y_Vehicle_CoorSys_E[m]_/1(Out1) -> Bus Creator1/6  "Pos_y_Vehicle_CoorSys_E[m]"
  Pos_x_Vehicle_CoorSys_E[m]_/1(Out1) -> Bus Creator1/5  "Pos_x_Vehicle_CoorSys_E[m]"
  Pos_x_Vehicle_CoorSys_E[m]/1 -> Pos_x_Vehicle_CoorSys_E[m]_/1(In1)
  v_y_Vehicle_CoG[km|h]/1 -> v_y_Vehicle[km|h]_/1(In1)
  v_x_Vehicle_CoG[km|h]/1 -> v_x_Vehicle[km|h]_/1(In1)
  Pos_y_Preview_Road[m]_/1(Out1) -> Bus Creator1/31  "Pos_y_Preview_Road[m]"
  Pos_x_Preview_Road[m]_/1(Out1) -> Bus Creator1/30  "Pos_x_Preview_Road[m]"
  Angle_Yaw_Veh_Road[deg]_/1(Out1) -> Bus Creator1/35  "Angle_Yaw_Veh_Road[deg]"
  Angle_Yaw_Veh_Road[deg]/1 -> Angle_Yaw_Veh_Road[deg]_/1(In1)
  Pos_x_Preview_Road[m]/1 -> Pos_x_Preview_Road[m]_/1(In1)
  Pos_y_Preview_Road[m]/1 -> Pos_y_Preview_Road[m]_/1(In1)
  i_Steering_Mean[]_/1(Out1) -> Bus Creator1/15  "i_Steering_Mean[]"
  CorneringStiffness_Tire_Rear[N|rad]_/1(Out1) -> Bus Creator1/14  "CorneringStiffness_Tire_Rear[N|rad]"
  CorneringStiffness_Tire_Front[N|rad]_/1(Out1) -> Bus Creator1/13  "CorneringStiffness_Tire_Front[N|rad]"
  Inertia_z_Vehicle_Total[kgm2]_/1(Out1) -> Bus Creator1/12  "Inertia_z_Vehicle_Total[kgm2]"
  YawRate_Vehicle[deg|s]_/1(Out1) -> Bus Creator1/8  "YawRate_Vehicle[deg|s]"
  Pos_x_CoG_Vehicle_Total[m]_/1(Out1) -> Bus Creator1/11  "Pos_x_CoG_Vehicle_Total[m]"
  Angle_Yaw_Vehicle_CoorSys_E[deg]_/1(Out1) -> Bus Creator1/7  "Angle_Yaw_Vehicle_CoorSys_E[deg]"
  i_Steering_Mean[]/1 -> i_Steering_Mean[]_/1(In1)
  CorneringStiffness_Tire_Rear[N|rad]/1 -> CorneringStiffness_Tire_Rear[N|rad]_/1(In1)
  CorneringStiffness_Tire_Front[N|rad]/1 -> CorneringStiffness_Tire_Front[N|rad]_/1(In1)
  Inertia_z_Vehicle_Total[kgm2]/1 -> Inertia_z_Vehicle_Total[kgm2]_/1(In1)
  YawRate_Vehicle[deg|s]/1 -> YawRate_Vehicle[deg|s]_/1(In1)
  Pos_x_CoG_Vehicle_Total[m]/1 -> Pos_x_CoG_Vehicle_Total[m]_/1(In1)
  v_y_Vehicle[km|h]_/1(Out1) -> Bus Creator1/4  "v_y_Vehicle[km|h]"
  s_Vehicle_Init[m]_/1(Out1) -> Bus Creator1/20  "s_Vehicle_Init[m]"
  s_Vehicle_Init[m]/1 -> s_Vehicle_Init[m]_/1(In1)
  Route_Direction_Init[]/1 -> Route_Direction_Init[]_/1(In1)
  Route_Direction_Init[]_/1(Out1) -> Bus Creator1/21  "Route_Direction_Init[]"
  Curv_Veh_Road[1|m]_/1(Out1) -> Bus Creator1/34  "Curv_Veh_Road[1|m]"
  Curv_Veh_Road[1|m]/1 -> Curv_Veh_Road[1|m]_/1(In1)
  Dist_Border_Left[m]_/1(Out1) -> Bus Creator1/32  "Dist_Border_Left[m]"
  Dist_Border_Right[m]_/1(Out1) -> Bus Creator1/33  "Dist_Border_Right[m]"
  Dist_Border_Left[m]/1 -> Dist_Border_Left[m]_/1(In1)
  Dist_Border_Right[m]/1 -> Dist_Border_Right[m]_/1(In1)
  s_Total_Vehicle_Road[m]_/1(Out1) -> Bus Creator1/22  "s_Total_Vehicle_Road[m]"
  Roll_Preview_Road[deg]_/1(Out1) -> Bus Creator1/26  "Roll_Preview_Road[deg]"
  Roll_Preview_Road[deg]/1 -> Roll_Preview_Road[deg]_/1(In1)
  Pos_y_Preview_DriverCurv[m]_/1(Out1) -> Bus Creator1/29  "Pos_y_Preview_DriverCurv[m]"
  Speed_Limit_Preview_Road[km|h]/1 -> Speed_Limit_Preview_Road[km|h]_/1(In1)
  Pos_x_Preview_DriverCurv[m]_/1(Out1) -> Bus Creator1/28  "Pos_x_Preview_DriverCurv[m]"
  Pos_z_Preview_Road[m]_/1(Out1) -> Bus Creator1/25  "Pos_z_Preview_Road[m]"
  Pitch_Preview_Road[deg]_/1(Out1) -> Bus Creator1/27  "Pitch_Preview_Road[deg]"
  Pitch_Preview_Road[deg]/1 -> Pitch_Preview_Road[deg]_/1(In1)
  Pos_z_Preview_Road[m]/1 -> Pos_z_Preview_Road[m]_/1(In1)
  Curv_Preview_Road[1|m]/1 -> Curv_Preview_Road[1|m]_/1(In1)
  s_Total_Vehicle_Road[m]/1 -> s_Total_Vehicle_Road[m]_/1(In1)
  Pos_x_Preview_DriverCurv[m]/1 -> Pos_x_Preview_DriverCurv[m]_/1(In1)
  Pos_y_Preview_DriverCurv[m]/1 -> Pos_y_Preview_DriverCurv[m]_/1(In1)
  Curv_Preview_Road[1|m]_/1(Out1) -> Bus Creator1/23  "Curv_Preview_Road[1|m]"
  Speed_Limit_Preview_Road[km|h]_/1(Out1) -> Bus Creator1/24  "Speed_Limit_Preview_Road[km|h]"
  State_Engine[0|1|2|3|4]_/1(Out1) -> Bus Creator1/18  "State_Engine[0|1|2|3|4]"
  State_Engine[0|1|2|3|4]/1 -> State_Engine[0|1|2|3|4]_/1(In1)
  State_StartStop[1Off|2NotReady|3Ready|4EngStopped]_/1(Out1) -> Bus Creator1/64  "State_StartStop[1Off|2NotReady|3Ready|4EngStopped]"
  State_StartStop[1Off|2NotReady|3Ready|4EngStopped]/1 -> State_StartStop[1Off|2NotReady|3Ready|4EngStopped]_/1(In1)
  omega_Out_Trm[rad|s]_/1(Out1) -> Bus Creator1/17  "omega_Out_Trm[rad|s]"
  omega_Out_Trm[rad|s]/1 -> omega_Out_Trm[rad|s]_/1(In1)
  m_Total_Vehicle[kg]/1 -> m_Total_Vehicle[kg]_/1(In1)
  n_Engine[rpm]/1 -> n_Engine[rpm]_/1(In1)
  n_Engine[rpm]_/1(Out1) -> Bus Creator1/16  "n_Engine[rpm]"
  v_x_Vehicle[km|h]_/1(Out1) -> Bus Creator1/3  "v_x_Vehicle[km|h]"
  Reset_States[0|1]_/1(Out1) -> Bus Creator1/19  "Reset_States[0|1]"
  Reset_States[0|1]/1 -> Reset_States[0|1]_/1(In1)
  F_Driving_Res[N]/1 -> F_Driving_Res[N]_/1(In1)
  Enable_v_Init[0|1]_/1(Out1) -> Bus Creator1/52  "Enable_v_Init[0|1]"
  Enable_v_Init[0|1]/1 -> Enable_v_Init[0|1]_/1(In1)
  Mode_AdaptVelocityToRoad[1Off|2On]_/1(Out1) -> Bus Creator1/59  "Mode_AdaptVelocityToRoad[1Off|2On]"
  Mode_LatCtrl[1Pos|2Yaw]_/1(Out1) -> Bus Creator1/58  "Mode_LatCtrl[1Pos|2Yaw]"
  Sw_LatDriver[1LatCtrl1|2LatCtrl2]_/1(Out1) -> Bus Creator1/57  "Sw_LatDriver[1LatCtrl1|2LatCtrl2]"
  Mode_Transmission[1Manual|2Automatic]_/1(Out1) -> Bus Creator1/53  "Mode_Transmission[1Manual|2Automatic]"
  Mode_AcceleratorBrake[1Stim|2Driver]_/1(Out1) -> Bus Creator1/54  "Mode_AcceleratorBrake[1Stim|2Driver]"
  Mode_GearClutch[1Stim|2Driver|3OpenClutch|4RefGear]/1 -> Mode_GearClutch[1Stim|2Driver|3OpenClutch|4RefGear]_/1(In1)
  Mode_AcceleratorBrake[1Stim|2Driver]/1 -> Mode_AcceleratorBrake[1Stim|2Driver]_/1(In1)
  Mode_Transmission[1Manual|2Automatic]/1 -> Mode_Transmission[1Manual|2Automatic]_/1(In1)
  Mode_GearClutch[1Stim|2Driver|3OpenClutch|4RefGear]_/1(Out1) -> Bus Creator1/55  "Mode_GearClutch[1Stim|2Driver|3OpenClutch|4RefGear]"
  Mode_CurvatureCalculation[1Road|2Driver]_/1(Out1) -> Bus Creator1/62  "Mode_CurvatureCalculation[1Road|2Driver]"
  Mode_ForceToRoad[1Off|2On]_/1(Out1) -> Bus Creator1/60  "Mode_ForceToRoad[1Off|2On]"
  Mode_ForceToRoad[1Off|2On]/1 -> Mode_ForceToRoad[1Off|2On]_/1(In1)
  Mode_CurvatureCalculation[1Road|2Driver]/1 -> Mode_CurvatureCalculation[1Road|2Driver]_/1(In1)
  Sw_LatDriver[1LatCtrl1|2LatCtrl2]/1 -> Sw_LatDriver[1LatCtrl1|2LatCtrl2]_/1(In1)
  Mode_SelectorLever[1Stim|2Driver]/1 -> Mode_SelectorLever[1Stim|2Driver]_/1(In1)
  Mode_Steer[1Stim|2Driver|3Fix]_/1(Out1) -> Bus Creator1/56  "Mode_Steer[1Stim|2Driver|3Fix]"
  Mode_SelectorLever[1Stim|2Driver]_/1(Out1) -> Bus Creator1/61  "Mode_SelectorLever[1Stim|2Driver]"
  Mode_TrafficDriver[1Off|2On]_/1(Out1) -> Bus Creator1/63  "Mode_TrafficDriver[1Off|2On]"
  Mode_TrafficDriver[1Off|2On]/1 -> Mode_TrafficDriver[1Off|2On]_/1(In1)
  Mode_AdaptVelocityToRoad[1Off|2On]/1 -> Mode_AdaptVelocityToRoad[1Off|2On]_/1(In1)
  Mode_LatCtrl[1Pos|2Yaw]/1 -> Mode_LatCtrl[1Pos|2Yaw]_/1(In1)
  Mode_Steer[1Stim|2Driver|3Fix]/1 -> Mode_Steer[1Stim|2Driver|3Fix]_/1(In1)
  n_Engine_Idle_Set[rpm]/1 -> n_Engine_Idle_Set[rpm]_/1(In1)
  n_Engine_Idle_Set[rpm]_/1(Out1) -> Bus Creator1/65  "n_Engine_Idle_Set[rpm]"
  Lane_ID_Vehicle[]/1 -> Lane_ID_Vehicle[]_/1(In1)
  Lane_ID_Vehicle[]_/1(Out1) -> Bus Creator1/66  "Lane_ID_Vehicle[]"

== system ASM_Traffic/Driver/Interface_Out/Plant_ModelSignals ==
  Pos_AccPedal[%] : Inport
  Pos_BrakePedal[%] : Inport  Port=2
  Pos_ClutchPedal[%] : Inport  Port=3
  Gear[] : Inport  Port=4
  SelectorLever[-3T|-2P|-1R|0N|1D] : Inport  Port=5
  s_Preview[m] : Inport  Port=6
  Angle_SteeringWheel[deg] : Inport  Port=7
  t_Preview_vRef_Driver[s] : Inport  Port=8
  Angle_SteeringWheel[deg]_ : Subsystem
      mask Display: disp('')
  Bus Creator : BusCreator  Inputs=8
  Gear[]_ : Subsystem
      mask Display: disp('')
  Pos_AccPedal[%]_ : Subsystem
      mask Display: disp('')
  Pos_BrakePedal[%]_ : Subsystem
      mask Display: disp('')
  Pos_ClutchPedal[%]_ : Subsystem
      mask Display: disp('')
  SelectorLever[-3T|-2P|-1R|0N|1D]_ : Subsystem
      mask Display: disp('')
  s_Preview[m]_ : Subsystem
      mask Display: disp('')
  t_Preview_vRef_Driver[s]_ : Subsystem
      mask Display: disp('')
  Out : Outport  VectorParamsAs1DForOutWhenUnconnected=off
  wires:
  s_Preview[m]_/1(Out1) -> Bus Creator/6  "s_Preview[m]"
  s_Preview[m]/1 -> s_Preview[m]_/1(In1)
  Angle_SteeringWheel[deg]_/1(Out1) -> Bus Creator/7  "Angle_SteeringWheel[deg]"
  Bus Creator/1 -> Out/1  "Plant"
  Angle_SteeringWheel[deg]/1 -> Angle_SteeringWheel[deg]_/1(In1)
  SelectorLever[-3T|-2P|-1R|0N|1D]_/1(Out1) -> Bus Creator/5  "SelectorLever[-3T|-2P|-1R|0N|1D]"
  SelectorLever[-3T|-2P|-1R|0N|1D]/1 -> SelectorLever[-3T|-2P|-1R|0N|1D]_/1(In1)
  Pos_AccPedal[%]_/1(Out1) -> Bus Creator/1  "Pos_AccPedal[%]"
  Pos_AccPedal[%]/1 -> Pos_AccPedal[%]_/1(In1)
  Gear[]/1 -> Gear[]_/1(In1)
  Gear[]_/1(Out1) -> Bus Creator/4  "Gear[]"
  Pos_ClutchPedal[%]/1 -> Pos_ClutchPedal[%]_/1(In1)
  Pos_ClutchPedal[%]_/1(Out1) -> Bus Creator/3  "Pos_ClutchPedal[%]"
  Pos_BrakePedal[%]_/1(Out1) -> Bus Creator/2  "Pos_BrakePedal[%]"
  Pos_BrakePedal[%]/1 -> Pos_BrakePedal[%]_/1(In1)
  t_Preview_vRef_Driver[s]/1 -> t_Preview_vRef_Driver[s]_/1(In1)
  t_Preview_vRef_Driver[s]_/1(Out1) -> Bus Creator/8  "t_Preview_vRef_Driver[s]"

== system ASM_Traffic/Driver/Plant/Driver ==
  UserInterface : Inport
  Interface_In : Inport  Port=2
  steering_wheel[deg] : Inport  Port=3
  ASMSignalCollector : Subsystem
  Angle_SW_Switch : Constant  Value=0
  COMMON_DRIVER_PARAMETERS : ASM_Environment_lib/Environment/Driver/COMMON_DRIVER_PARAMETERS  Tag=ASM_SUBCOMPONENT  Const_Angle_Max_SteeringWheel=MDL.Environment.Driver.Const_Angle_Max_SteeringWheel  ASMProperties=struct('Name','COMMON_DRIVER_PARAMETERS','Version','3.0','Library','ASM_Environment_lib')  ASMInstanceName=common_driver_parameters  ASMInstanceID=1
  Goto Tag Visibility1 : GotoTagVisibility  GotoTag=ASMBUS_Driver_OutputSignals
  Goto Tag Visibility2 : GotoTagVisibility  GotoTag=ASMBUS_Driver_LongCtrl
  Goto Tag Visibility3 : GotoTagVisibility  GotoTag=ASMBUS_Driver_GearShifter
  Goto Tag Visibility4 : GotoTagVisibility  GotoTag=ASMBUS_Driver_LatCtrl1
  Goto Tag Visibility5 : GotoTagVisibility  GotoTag=ASMBUS_Driver_LatCtrl2
  Goto Tag Visibility6 : GotoTagVisibility  GotoTag=ASMBUS_Driver_LatCtrl_PosError
  Goto Tag Visibility7 : GotoTagVisibility  GotoTag=ASMBUS_Driver_SpeedProfiler
  Goto Tag Visibility8 : GotoTagVisibility  GotoTag=ASMBUS_Driver_Curvature
  LateralController : Subsystem
  LongitudinalController : Subsystem
  ModelDesk_MC_ID_Environment : ASM_Utils_lib/ModelDeskInterface/ModelDesk_MC  Tag=ASM_MAINCOMPONENT  Editable=off  MainComponent=Environment
  OutputSignals : Subsystem
  ReferenceVelocity : Subsystem
  Switch : Switch  Criteria=u2 ~= 0  SaturateOnIntegerOverflow=off  InputSameDT=off
  Terminator : Terminator
  ASMSignalBus : Outport  VectorParamsAs1DForOutWhenUnconnected=off
  wires:
  LateralController/2(Angle_SteeringWheel[deg]) -> Switch/1
  LateralController/1(s_Preview_LatCtrl[m]) -> OutputSignals/7(s_Preview_LatCtrl[m])
  ReferenceVelocity/3(s_Preview_vRef[m]) -> OutputSignals/6(s_Preview_vRef[m])
  ReferenceVelocity/2(v_Vehicle_Ref_Preview[m|s]) -> LongitudinalController/3(v_Vehicle_Ref_Preview[m|s])
  ReferenceVelocity/1(v_Vehicle_Ref[m|s]) -> LongitudinalController/2(v_Vehicle_Ref[m|s])
  LongitudinalController/1(t_Preview_vRef[s]) -> ReferenceVelocity/2(t_Preview_vRef[s])
  ASMSignalCollector/1(ASMSignalBus) -> ASMSignalBus/1
  Interface_In/1 -> LongitudinalController/1(Interface_In), ReferenceVelocity/1(Interface_In), LateralController/1(Interface_In)
  LongitudinalController/2(Pos_AccPedal[%]) -> OutputSignals/1(Pos_AccPedal[%])
  LongitudinalController/6(SelectorLever[-3T|-2P|-1R|0N|1D]) -> OutputSignals/5(SelectorLever[-3T|-2P|-1R|0N|1D])
  LongitudinalController/4(Pos_ClutchPedal[%]) -> OutputSignals/3(Pos_ClutchPedal[%])
  LongitudinalController/3(Pos_BrakePedal[%]) -> OutputSignals/2(Pos_BrakePedal[%])
  LongitudinalController/5(Gear[]) -> OutputSignals/4(Gear[])
  UserInterface/1 -> Terminator/1
  Angle_SW_Switch/1 -> Switch/2
  steering_wheel[deg]/1 -> Switch/3
  Switch/1 -> OutputSignals/8(Angle_SteeringWheel[deg])

== system ASM_Traffic/Driver/Plant/UserInterface ==
  note: Driver
  In : Inport
  Interface_In : Inport  Port=2
  ASMSignalBus_Plant : Subsystem
  DISP_Plant : Subsystem
  PAR_Plant : Subsystem
  Out : Outport  VectorParamsAs1DForOutWhenUnconnected=off
  wires:
  In/1 -> DISP_Plant/2(In), ASMSignalBus_Plant/1(In)
  PAR_Plant/1(Out) -> Out/1
  Interface_In/1 -> DISP_Plant/1(Interface_In)

== system ASM_Traffic/Driver/SignalInterface/ASMSignalInterface ==
  ASMSignalBus : Inport
  Enable : EnablePort
  signal_structure : Subsystem
  wires:
  ASMSignalBus/1 -> signal_structure/1(ASMSignalBus)

== system ASM_Traffic/Driver/SignalInterface/ExternalOutports ==
  In1 : Inport
  Enable : EnablePort
  Driver : dsmpblib/Data Outport  Tag=ASM_MPB  Priority=-10000
      settings: SourceProductName=dSPACE Model Interface Package for Simulink (MIPS)
  Select_Outport_Signals : Subsystem
  wires:
  In1/1 -> Select_Outport_Signals/1(ASMSignalBus)
  Select_Outport_Signals/9(a_y_Ref[m|s2]) -> Driver/9
  Select_Outport_Signals/8(a_x_Ref[m|s2]) -> Driver/8
  Select_Outport_Signals/7(v_x_Ref[km|h]) -> Driver/7
  Select_Outport_Signals/6(Angle_SteeringWheel[deg]) -> Driver/6
  Select_Outport_Signals/5(SelectorLever[-3T|-2P|-1R|0N|1D]) -> Driver/5
  Select_Outport_Signals/4(Gear[]) -> Driver/4
  Select_Outport_Signals/3(Pos_ClutchPedal[%]) -> Driver/3
  Select_Outport_Signals/2(Pos_BrakePedal[%]) -> Driver/2
  Select_Outport_Signals/1(Pos_AccPedal[%]) -> Driver/1
